simulink model "AvonGasTurbineDgTwin_fixed"  (R2024b)
settings: Solver=VariableStepAuto  StartTime=0  StopTime=7200  FixedStep=1  RelTol=1e-3  EnableMultiTasking=on
InitFcn:
  | warning off
model workspace (MAT data in the model file):
  FAULT_01_AirIntakeFilterFouling_enable = 1
  FAULT_02_CompBladeFouling_enable = 1
  FAULT_03_CompBladeDamage_enable = 1
  FAULT_04_CompSurgeStall_enable = 1
  FAULT_05_DiffuserDamage_enable = 1
  FAULT_06_IGVStuck_enable = 1
  FAULT_07_FuelPrssRegulatorStuck_enable = 1
  FAULT_08_FuelValveLeakage_enable = 1
  FAULT_09_FuelContamination_enable = 1
  FAULT_10_FuelLineBlockage_enable = 1
  FAULT_11_FuelPumpDegradation_enable = 1
  FAULT_12_FuelSupplyPressDrop_enable = 1
  FAULT_13_FGSupplyPressOscillation_enable = 1
  FAULT_14_FGValvePartialOpening_enable = 1
  FAULT_15_FGValveActuatorDelay_enable = 1
  FAULT_15_FuelPressReg_enable = 0
  FAULT_16_CombLinerDamage_enable = 1
  FAULT_16_FuelValveLeak_enable = 0
  FAULT_17_FuelNozzleClogging_enable = 1
  FAULT_18_CombustionFlameOscillation_enable = 1
  FAULT_19_CombustionInstability_enable = 1
  FAULT_20_HotGasPathTempIncrease_enable = 1
  FAULT_21_GGTurbFouling_enable = 1
  FAULT_22_GGTurbBladeDamage_enable = 1
  FAULT_23_GGNozzleBlockage_enable = 1
  FAULT_24_GGSealDegradation_enable = 1
  FAULT_25_GGInletPressureLoss_enable = 1
  FAULT_26_PTFouling_enable = 1
  FAULT_27_PTBladeDamage_enable = 1
  FAULT_28_PTNozzleDamage_enable = 1
  FAULT_29_PTSealDegradation_enable = 1
  FAULT_30_PTBearingWear_enable = 1
  FAULT_31_PTPowerLoss_enable = 1
  FAULT_32_PTStackBlockage_enable = 1
  FAULT_33_SensorEnhancement_enable = 1
  FAULT_34_SensorDegradation_enable = 1
  FAULT_35_SensorEnhanceStep_enable = 1
  FAULT_36_SensorDegradeStep_enable = 1
  FAULT_37_SensorFreez_enable = 1
  FAULT_38_GGSpeedSensor_enable = 1
  FAULT_39_PTSpeedSensor_enable = 1
  FAULT_40_FGSensorOffset_enable = 1
  FAULT_41_FGSensorDrift_enable = 1
  FAULT_42_ControlLoopOscillation_enable = 1
  GOV_GG_BASELINE = 10
  GOV_GG_DROOP_PCT = 0.04
  GOV_PT_BASELINE = 10
  GOV_PT_DROOP_PCT = 0.04
  SW_Manual_Switch1_enable = 1
  SW_Manual_Switch2_enable = 1
  SW_Manual_Switch3_enable = 1
  SW_Manual_Switch4_enable = 1
  SW_Manual_Switch_enable = 1
undefined symbols (not defined in the file or in its folder): ENV_ambient_moisture_pct, ENV_comp_inlet_press_kPa, ENV_FG_pressure_kPa, ENV_FG_temp_C, SP_POWER_CMD
libraries: slpidlib x3, simulink x2
(part 3 of 4)

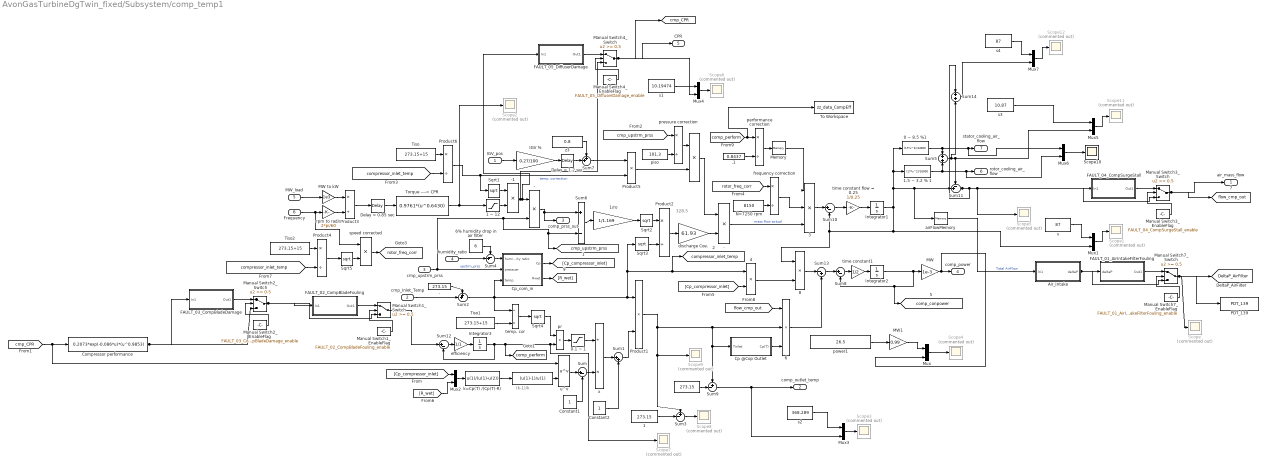
== system AvonGasTurbineDgTwin_fixed/Subsystem/comp_temp1 ==
  note: (k-1)/k
  note: 328.5
  IGV_pos : Inport
  cmp_Inlet_Temp : Inport  Port=2
  cmp_upstrm_prss : Inport  Port=3
  humidity_ratio : Inport  Port=4
  MW_load : Inport  Port=5
  Frequency : Inport  Port=6
  " " : Fcn  Expr=(u(1)-1)/u(1)
  "    " : Constant  Value=273.15
  "     " : Product  RndMeth=Zero
  "    1" : Constant  Value=273.15
  " 1.5 ~ 3.2 % 1" : Fcn  Expr=(17*u^2)/16000  SampleTime=1
  " 3" : Product  Inputs=3  RndMeth=Zero
  " 4" : Product  RndMeth=Zero
  " 6" : Product  Inputs=3  RndMeth=Zero
  " 8" : Product  RndMeth=Zero
  - : Product  RndMeth=Zero
  -1 : Product  RndMeth=Zero
  . : Constant  Value=273.15
  ". " : Product  RndMeth=Zero
  .1 : Constant  Value=0.8437
  0 ~ 8.5 %1 : Fcn  Expr=(17*u^2)/44000  SampleTime=1
  0.1 ~ 1 : Saturate  UpperLimit=1  LowerLimit=0.1
  1 ~ 12 : Saturate  UpperLimit=20  LowerLimit=1
  1/ro : Gain  Gain=1/1.169
  6% humidity drop in air filter : Constant  Value=6
  Air_Intake : Subsystem
  "Compressor performance " : Fcn  Expr=0.2073*exp(-0.086*u)*(u^0.9853)
  Constant1 : Constant
  Constant2 : Constant
  Cp @Cop Outlet : Subsystem
  Cp_com_in : Subsystem
  Delay = 0.85 sec : TransportDelay  DelayTime=0.85  InitialOutput=10.706
  Delay = 1.2 sec : TransportDelay  DelayTime=1.2  InitialOutput=0.27
  FAULT_01_AirIntakeFilterFouling : Subsystem
  FAULT_02_CompBladeFouling : Subsystem
  FAULT_03_CompBladeDamage : Subsystem
  FAULT_04_CompSurgeStall : Subsystem
  FAULT_05_DiffuserDamage : Subsystem
  IGV % : Gain  Gain=0.27/100
  Integrator1 : Integrator  InitialCondition=87  LimitOutput=on  UpperSaturationLimit=140  LowerSaturationLimit=1
  Integrator2 : Integrator  InitialCondition=28000  LimitOutput=on  UpperSaturationLimit=32000  LowerSaturationLimit=10
  Integrator3 : Integrator  InitialCondition=0.6  LimitOutput=on  UpperSaturationLimit=1  LowerSaturationLimit=0
  MW : Gain  Gain=1e-3
  MW to kW : Gain  Gain=1e3
  MW1 : Gain  Gain=0.99
  Manual Switch1_EnableFlag : Constant  Value=FAULT_02_CompBladeFouling_enable
  Manual Switch1_Switch : Switch  Threshold=0.5  SaturateOnIntegerOverflow=off  InputSameDT=off
  Manual Switch2_EnableFlag : Constant  Value=FAULT_03_CompBladeDamage_enable
  Manual Switch2_Switch : Switch  Threshold=0.5  SaturateOnIntegerOverflow=off  InputSameDT=off
  Manual Switch3_EnableFlag : Constant  Value=FAULT_04_CompSurgeStall_enable
  Manual Switch3_Switch : Switch  Threshold=0.5  SaturateOnIntegerOverflow=off  InputSameDT=off
  Manual Switch4_EnableFlag : Constant  Value=FAULT_05_DiffuserDamage_enable
  Manual Switch4_Switch : Switch  Threshold=0.5  SaturateOnIntegerOverflow=off  InputSameDT=off
  Manual Switch7_EnableFlag : Constant  Value=FAULT_01_AirIntakeFilterFouling_enable
  Manual Switch7_Switch : Switch  Threshold=0.5  SaturateOnIntegerOverflow=off  InputSameDT=off
  Memory : Memory  InitialCondition=1.5
  Mux{,1..7} (8 alike) : Mux  Inputs=2
  N=7250 rpm : Constant  Value=8150
  PDT_139 : ToWorkspace  VariableName=PDT_139  SampleTime=0.2
  Product1 : Product  RndMeth=Zero
  Product{2..4,6} (4 alike) : Product  Inputs=*/  RndMeth=Zero
  Product5 : Product  RndMeth=Zero
  Scope{,1..9,11..12} (12 alike) : Scope  Commented=on
  Scope10 : Scope
  Sqrt{1..5} (5 alike) : Sqrt
  Sum{,8,10,12} (4 alike) : Sum  Inputs=|+-
  Sum1 : Sum  Inputs=|++
  Sum11 : Sum  Inputs=-+|
  Sum13 : Sum  Inputs=|-+
  Sum14 : Sum
  Sum2 : Sum  Inputs=++|
  Sum3 : Sum  Inputs=+-|
  Sum4 : Sum  Inputs=-+|
  Sum5 : Sum
  Sum6 : Sum  Inputs=+-
  Sum7 : Sum  Inputs=++|
  Sum9 : Sum  Inputs=+-|
  Tiso : Constant  Value=273.15+15
  Tiso1 : Constant  Value=273.15+15
  Tiso2 : Constant  Value=273.15+15
  To Workspace : ToWorkspace  VariableName=zz_data_CompEff  SampleTime=0.2
  Torque ----> CPR : Fcn  Expr=0.9761*(u^0.6430)
  airFlowMemory : Memory  InitialCondition=80
  "discharge Coe. " : Gain  Gain=61.93
  efficiency : Gain  Gain=1/1
  frequency correction : Product  Inputs=*/  RndMeth=Zero
  k=Cp(T) /(Cp(T)-R) : Fcn  Expr=u(1)/(u(1)-u(2))
  performance correction : Product  Inputs=*/  RndMeth=Zero
  piso : Constant  Value=101.3
  power1 : Constant  Value=26.5
  "pr " : Product  RndMeth=Zero
  pressure correction : Product  Inputs=*/  RndMeth=Zero
  rpm to rad/s : Gain  Gain=2*pi/60
  s : Constant  Value=87
  s1 : Constant  Value=10.19474
  s2 : Constant  Value=368.289
  s3 : Constant  Value=10.87
  s4 : Constant  Value=87
  speed corrected : Product  RndMeth=Zero
  temp. cor : Product  Inputs=/*  RndMeth=Zero
  time constant flow = 0.25 : Gain  Gain=1/0.25
  time constant1 : Gain  Gain=1/2
  u^v : Math  Operator=pow  SignedPower=on
  x : Product  Inputs=/*  RndMeth=Zero
  z3 : Constant  Value=0.8
  air_mass_flow : Outport
  comp_outlet_temp : Outport  Port=2
  comp_prss_out : Outport  Port=3
  comp_power : Outport  Port=4
  CPR : Outport  Port=5
  rotor_cooling_air_flow : Outport  Port=6
  stator_cooling_air_flow : Outport  Port=7
  tag scope: DeltaP_AirFilter=global, cmp_CPR=global, cmp_upstrm_prss=global, comp_conpower=global, comp_perform=global, compressor_inlet_temp=global, flow_cmp_out=global, rotor_freq_corr=global
  wires:
  [cmp_CPR] -> "Compressor performance "/1, u^v/1
  " "/1 -> u^v/2
  u^v/1 -> Sum/1
  Sum/1 -> x/2
  Constant2/1 -> Sum1/2
  Sum1/1 -> Product1/2
  Sum2/1 -> Cp_com_in/3(temp.), Product1/1, Sqrt3/1, [compressor_inlet_temp], " 4"/1, temp. cor/1
  x/1 -> Sum1/1
  Constant1/1 -> Sum/2
  cmp_upstrm_prss/1 -> Cp_com_in/2(pressuer), -/2, [cmp_upstrm_prss], Sum6/2  "upstrm_prss"
  cmp_Inlet_Temp/1 -> Sum2/2
  0.1 ~ 1/1 -> x/1
  k=Cp(T) /(Cp(T)-R)/1 -> " "/1
  Cp_com_in/1(Cp) -> [Cp_compressor_inlet]
  Sum4/1 -> Cp_com_in/1(humidity ratio)
  humidity_ratio/1 -> Sum4/2
  6% humidity drop in air filter/1 -> Sum4/1
  -/1 -> comp_prss_out/1, Sum6/1
  Frequency/1 -> speed corrected/1, rpm to rad/s/1
  Sum6/1 -> 1/ro/1
  1/ro/1 -> Sqrt2/1
  Sqrt3/1 -> Product2/2
  Product2/1 -> "discharge Coe. "/1
  Sqrt2/1 -> Product2/1
  IGV_pos/1 -> IGV %/1
  piso/1 -> pressure correction/2
  [cmp_upstrm_prss] -> pressure correction/1
  Product5/1 -> "     "/2
  "discharge Coe. "/1 -> ". "/2
  "     "/1 -> ". "/1
  ". "/1 -> " 3"/3  "mass flow actual"
  Product6/1 -> Product5/2, Sqrt1/1  "temp. correction"
  Tiso/1 -> Product6/1
  [compressor_inlet_temp] -> Product6/2
  pressure correction/1 -> "     "/1
  1 ~ 12/1 -> -1/2
  N=7250 rpm/1 -> frequency correction/2
  [rotor_freq_corr] -> frequency correction/1
  frequency correction/1 -> " 3"/2
  " 3"/1 -> Sum10/1
  [Cp_compressor_inlet] -> " 4"/2
  Sum10/1 -> time constant flow = 0.25/1
  time constant flow = 0.25/1 -> Integrator1/1
  " 4"/1 -> " 8"/2
  " 8"/1 -> Sum13/1
  Sqrt1/1 -> -1/1
  Sum7/1 -> Product5/1
  z3/1 -> Sum7/1
  IGV %/1 -> Delay = 1.2 sec/1
  Delay = 1.2 sec/1 -> Sum7/2
  MW_load/1 -> MW to kW/1
  Cp_com_in/2(Rwet) -> [R_wet]
  Mux2/1 -> k=Cp(T) /(Cp(T)-R)/1
  [Cp_compressor_inlet] -> Mux2/1
  [R_wet] -> Mux2/2
  Sum8/1 -> time constant1/1
  time constant1/1 -> Integrator2/1
  Sum13/1 -> Sum8/1
  ./1 -> Sum2/1
  Tiso1/1 -> temp. cor/2
  temp. cor/1 -> Sqrt4/1
  "pr "/1 -> 0.1 ~ 1/1
  Sum12/1 -> efficiency/1
  efficiency/1 -> Integrator3/1
  Sqrt4/1 -> "pr "/1
  Torque ----> CPR/1 -> Scope2/1, 1 ~ 12/1
  MW to kW/1 -> Product3/1
  rpm to rad/s/1 -> Product3/2
  Integrator3/1 -> [comp_perform], Scope7/1, "pr "/2, Sum12/2
  Integrator2/1 -> MW/1, [comp_conpower], Sum8/2
  Product1/1 -> " 6"/2, Cp @Cop Outlet/1(Tinlet), Sum9/1, Scope9/1, Sum3/1
  Cp @Cop Outlet/1(Cp(T)) -> " 6"/3
  " 6"/1 -> Sum13/2
  "    "/1 -> Sum9/2
  Tiso2/1 -> Product4/1
  [compressor_inlet_temp] -> Product4/2
  speed corrected/1 -> [rotor_freq_corr]
  Product4/1 -> Sqrt5/1
  Sqrt5/1 -> speed corrected/2
  [flow_cmp_out] -> " 6"/1
  Mux/1 -> Scope4/1
  Sum11/1 -> Sum14/1, Scope5/1, FAULT_04_CompSurgeStall/1(In1), Manual Switch3_Switch/3
  0 ~ 8.5 %1/1 -> Sum5/1, Mux6/1, stator_cooling_air_flow/1
  Integrator1/1 -> Mux1/2, " 8"/1, Sum10/2, airFlowMemory/1, Sum11/2, " 1.5 ~ 3.2 % 1"/1, 0 ~ 8.5 %1/1
  Mux1/1 -> Scope1/1
  s/1 -> Mux1/1
  Product3/1 -> Delay = 0.85 sec/1
  Delay = 0.85 sec/1 -> Torque ----> CPR/1
  power1/1 -> MW1/1
  Mux3/1 -> Scope3/1
  s2/1 -> Mux3/1
  MW/1 -> Mux/2, comp_power/1
  Mux4/1 -> Scope6/1
  s1/1 -> Mux4/1
  -1/1 -> -/1, FAULT_05_DiffuserDamage/1(In1), Manual Switch4_Switch/3
  Sum9/1 -> Mux3/2, comp_outlet_temp/1
  "    1"/1 -> Sum3/2
  Sum3/1 -> Scope8/1
  MW1/1 -> Mux/1
  Sum5/1 -> Sum14/2, Sum11/1, Mux5/2
  Mux5/1 -> Scope11/1
  s3/1 -> Mux5/1
  Mux6/1 -> Scope10/1
  " 1.5 ~ 3.2 % 1"/1 -> Sum5/2, Mux6/2, rotor_cooling_air_flow/1
  Sum14/1 -> Mux7/2
  Mux7/1 -> Scope12/1
  s4/1 -> Mux7/1
  performance correction/1 -> Memory/1
  .1/1 -> performance correction/2
  [comp_perform] -> To Workspace/1, performance correction/1
  Memory/1 -> " 3"/1
  "Compressor performance "/1 -> FAULT_03_CompBladeDamage/1(In1), Manual Switch2_Switch/3
  airFlowMemory/1 -> Air_Intake/1(In1)  "Total AirFlow"
  Air_Intake/1(deltaP) -> FAULT_01_AirIntakeFilterFouling/1(deltaP), Manual Switch7_Switch/3
  FAULT_02_CompBladeFouling/1(Out1) -> Manual Switch1_Switch/1
  Manual Switch1_EnableFlag/1 -> Manual Switch1_Switch/2
  Manual Switch1_Switch/1 -> Sum12/1
  FAULT_03_CompBladeDamage/1(Out1) -> Manual Switch2_Switch/1
  Manual Switch2_EnableFlag/1 -> Manual Switch2_Switch/2
  Manual Switch2_Switch/1 -> Manual Switch1_Switch/3, FAULT_02_CompBladeFouling/1(In1)
  FAULT_04_CompSurgeStall/1(Out1) -> Manual Switch3_Switch/1
  Manual Switch3_EnableFlag/1 -> Manual Switch3_Switch/2
  Manual Switch3_Switch/1 -> air_mass_flow/1, [flow_cmp_out]
  FAULT_05_DiffuserDamage/1(Out1) -> Manual Switch4_Switch/1
  Manual Switch4_EnableFlag/1 -> Manual Switch4_Switch/2
  Manual Switch4_Switch/1 -> [cmp_CPR], CPR/1, Mux4/2
  FAULT_01_AirIntakeFilterFouling/1(Out1) -> Manual Switch7_Switch/1
  Manual Switch7_EnableFlag/1 -> Manual Switch7_Switch/2
  Manual Switch7_Switch/1 -> [DeltaP_AirFilter], PDT_139/1, Scope/1

== system AvonGasTurbineDgTwin_fixed/Subsystem2/FAULT_42_ControlLoopOscillation ==
  In1 : Inport
  FAULT_42_multiplier : FromWorkspace  VariableName=FAULT_42_multiplier  SampleTime=-1
  Mux : Mux  Inputs=2
  Product : Product
  Scope{,1..3} (4 alike) : Scope  Commented=on
  Out1 : Outport
  wires:
  FAULT_42_multiplier/1 -> Product/1, Scope/1
  In1/1 -> Scope1/1, Mux/2, Product/2
  Product/1 -> Mux/1, Scope2/1, Out1/1
  Mux/1 -> Scope3/1

== system AvonGasTurbineDgTwin_fixed/Subsystem/Combustor1/FAULT_16_CombLinerDamage ==
  air_flow : Inport
  FAULT_16_multiplier : FromWorkspace  VariableName=FAULT_16_multiplier  SampleTime=-1
  Mux : Mux  Inputs=2
  Product : Product
  Scope{,1..3} (4 alike) : Scope  Commented=on
  Out1 : Outport
  wires:
  FAULT_16_multiplier/1 -> Product/1, Scope/1
  air_flow/1 -> Scope1/1, Mux/2, Product/2
  Product/1 -> Mux/1, Scope2/1, Out1/1
  Mux/1 -> Scope3/1

== system AvonGasTurbineDgTwin_fixed/Subsystem/Combustor1/FAULT_17_FuelNozzleClogging ==
  FG flow : Inport
  FAULT_17_multiplier : FromWorkspace  VariableName=FAULT_17_multiplier  SampleTime=-1
  Mux : Mux  Inputs=2
  Product : Product
  Scope{,1..3} (4 alike) : Scope  Commented=on
  Out1 : Outport
  wires:
  FAULT_17_multiplier/1 -> Product/1, Scope/1
  FG flow/1 -> Scope1/1, Mux/2, Product/2
  Product/1 -> Mux/1, Scope2/1, Out1/1
  Mux/1 -> Scope3/1

== system AvonGasTurbineDgTwin_fixed/Subsystem/Combustor1/FAULT_18_CombustionFlameOscillation ==
  temp chamber 1 : Inport
  FAULT_18_multiplier : FromWorkspace  VariableName=FAULT_18_multiplier  SampleTime=-1
  Mux : Mux  Inputs=2
  Product : Product
  Scope{,1..3} (4 alike) : Scope  Commented=on
  Out1 : Outport
  wires:
  FAULT_18_multiplier/1 -> Product/1, Scope/1
  temp chamber 1/1 -> Scope1/1, Mux/2, Product/2
  Product/1 -> Mux/1, Scope2/1, Out1/1
  Mux/1 -> Scope3/1

== system AvonGasTurbineDgTwin_fixed/Subsystem/Combustor1/FAULT_19_CombustionInstability ==
  In1 : Inport
  FAULT_19_multiplier : FromWorkspace  VariableName=FAULT_19_multiplier  SampleTime=-1
  Mux : Mux  Inputs=2
  Product : Product
  Scope{,1..3} (4 alike) : Scope  Commented=on
  Out1 : Outport
  wires:
  FAULT_19_multiplier/1 -> Product/1, Scope/1
  In1/1 -> Scope1/1, Mux/2, Product/2
  Product/1 -> Mux/1, Scope2/1, Out1/1
  Mux/1 -> Scope3/1

== system AvonGasTurbineDgTwin_fixed/Subsystem/Combustor1/FAULT_20_HotGasPathTempIncrease ==
  In1 : Inport
  FAULT_20_multiplier : FromWorkspace  VariableName=FAULT_20_multiplier  SampleTime=-1
  Mux : Mux  Inputs=2
  Product : Product
  Scope{,1..3} (4 alike) : Scope  Commented=on
  Out1 : Outport
  wires:
  FAULT_20_multiplier/1 -> Product/1, Scope/1
  In1/1 -> Scope1/1, Mux/2, Product/2
  Product/1 -> Mux/1, Scope2/1, Out1/1
  Mux/1 -> Scope3/1

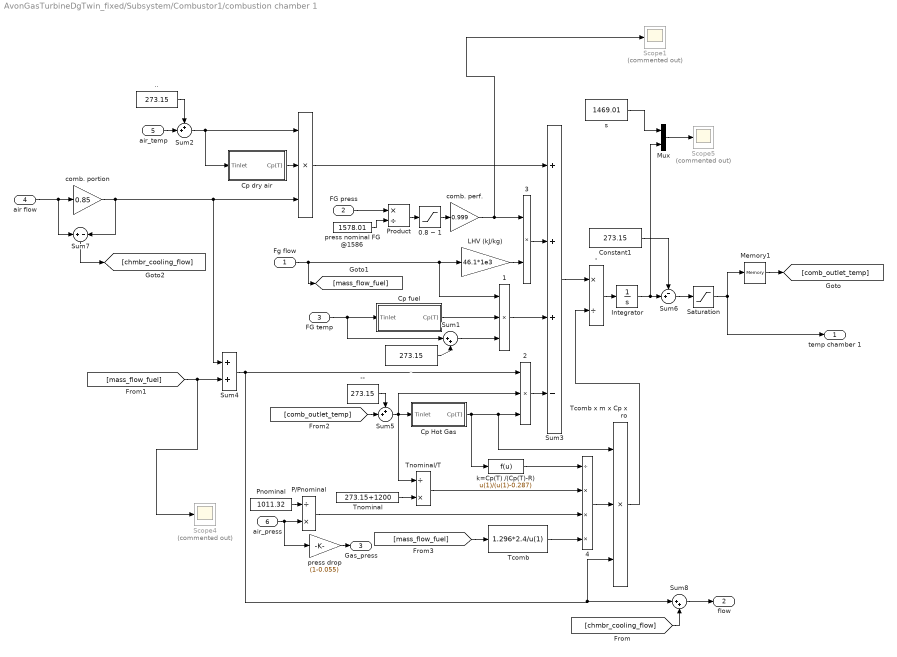
== system AvonGasTurbineDgTwin_fixed/Subsystem/Combustor1/combustion chamber 1 ==
  Fg flow : Inport
  FG press : Inport  Port=2
  FG temp : Inport  Port=3
  air flow : Inport  Port=4
  air_temp : Inport  Port=5
  air_press : Inport  Port=6
  "     " : Product  Inputs=3  RndMeth=Zero
  "     1" : Product  Inputs=3  RndMeth=Zero
  "     2" : Product  Inputs=3  RndMeth=Zero
  "     3" : Product  RndMeth=Zero
  "     4" : Product  Inputs=/***  RndMeth=Zero
  " Cp dry air " : Subsystem
  - : Product  Inputs=*/  RndMeth=Zero
  -- : Constant  Value=273.15
  . : Constant  Value=273.15
  .. : Constant  Value=273.15
  0.8 ~ 1 : Saturate  UpperLimit=1  LowerLimit=0.8
  Constant1 : Constant  Value=273.15
  "Cp Hot Gas " : Subsystem
  Cp fuel : Subsystem
  Integrator : Integrator  InitialCondition=780+273.15  LimitOutput=on  UpperSaturationLimit=2000  LowerSaturationLimit=780+273.15
  "LHV (kJ/kg) " : Gain  Gain=46.1*1e3
  Memory1 : Memory  InitialCondition=780
  Mux : Mux  Inputs=2
  P/Pnominal : Product  Inputs=/*  RndMeth=Zero
  Pnominal : Constant  Value=1011.32
  Product : Product  Inputs=*/
  Saturation : Saturate  UpperLimit=1400  LowerLimit=350
  Scope1 : Scope  Commented=on
  Scope4 : Scope  Commented=on
  Scope5 : Scope  Commented=on
  Sum1 : Sum  Inputs=|++
  Sum2 : Sum  Inputs=++|
  Sum3 : Sum  Inputs=+++-
  Sum4 : Sum  Inputs=2
  Sum5 : Sum  Inputs=++|
  Sum6 : Sum  Inputs=-+|
  Sum7 : Sum  Inputs=+-
  Sum8 : Sum  Inputs=|++
  Tcomb : Fcn  Expr=1.296*2.4/u(1)  SampleTime=1
  Tcomb x m x Cp x ro : Product  Inputs=3  RndMeth=Zero
  Tnominal : Constant  Value=273.15+1200
  Tnominal/T : Product  Inputs=/*  RndMeth=Zero
  comb. perf. : Gain  Gain=0.999
  comb. portion : Gain  Gain=0.85
  k=Cp(T) /(Cp(T)-R) : Fcn  Expr=u(1)/(u(1)-0.287)
  press drop : Gain  Gain=(1-0.055)  SampleTime=1
  press nominal FG @1586 : Constant  Value=1578.01
  s : Constant  Value=1469.01
  temp chamber 1 : Outport
  flow : Outport  Port=2
  Gas_press : Outport  Port=3
  wires:
  " Cp dry air "/1(Cp(T)) -> "     "/2
  ../1 -> Sum2/1
  Sum2/1 -> " Cp dry air "/1(Tinlet), "     "/1
  FG press/1 -> Product/1
  FG temp/1 -> Sum1/1, Cp fuel/1(Tinlet)
  Sum3/1 -> -/1
  Fg flow/1 -> "     1"/1, "LHV (kJ/kg) "/1, [mass_flow_fuel]
  Sum1/1 -> "     1"/3
  Cp fuel/1(Cp(T)) -> "     1"/2
  "     "/1 -> Sum3/1
  Memory1/1 -> [comb_outlet_temp]
  "     1"/1 -> Sum3/3
  ./1 -> Sum1/2
  "     2"/1 -> Sum3/4
  Tnominal/1 -> Tnominal/T/2
  Sum5/1 -> "     2"/2, "Cp Hot Gas "/1(Tinlet), Tnominal/T/1
  Constant1/1 -> Sum6/1
  Integrator/1 -> Mux/2, Sum6/2
  Sum6/1 -> Saturation/1
  "LHV (kJ/kg) "/1 -> "     3"/2
  Tcomb x m x Cp x ro/1 -> -/2
  Tnominal/T/1 -> "     4"/2
  [mass_flow_fuel] -> Scope4/1, Sum4/2
  "Cp Hot Gas "/1(Cp(T)) -> k=Cp(T) /(Cp(T)-R)/1, "     2"/3, Tcomb x m x Cp x ro/1
  --/1 -> Sum5/1
  Pnominal/1 -> P/Pnominal/1
  air_press/1 -> press drop/1, P/Pnominal/2
  "     4"/1 -> Tcomb x m x Cp x ro/2
  k=Cp(T) /(Cp(T)-R)/1 -> "     4"/1
  [comb_outlet_temp] -> Sum5/2
  P/Pnominal/1 -> "     4"/3
  air_temp/1 -> Sum2/2
  -/1 -> Integrator/1
  Saturation/1 -> temp chamber 1/1, Memory1/1
  s/1 -> Mux/1
  Sum4/1 -> "     2"/1, Sum8/1, Tcomb x m x Cp x ro/3
  Mux/1 -> Scope5/1
  press drop/1 -> Gas_press/1
  press nominal FG @1586/1 -> Product/2
  Product/1 -> 0.8 ~ 1/1
  0.8 ~ 1/1 -> comb. perf./1
  comb. perf./1 -> "     3"/1, Scope1/1
  "     3"/1 -> Sum3/2
  [mass_flow_fuel] -> Tcomb/1
  Tcomb/1 -> "     4"/4
  air flow/1 -> Sum7/1, comb. portion/1
  comb. portion/1 -> Sum7/2, "     "/3, Sum4/1
  Sum8/1 -> flow/1
  [chmbr_cooling_flow] -> Sum8/2
  Sum7/1 -> [chmbr_cooling_flow]

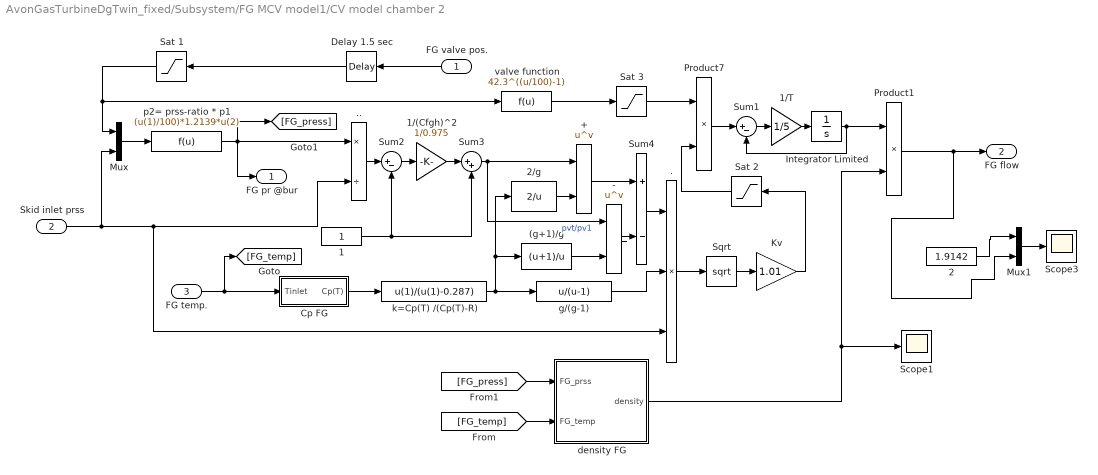
== system AvonGasTurbineDgTwin_fixed/Subsystem/FG MCV model1/CV model chamber 2 ==
  FG valve pos. : Inport
  Skid inlet prss : Inport  Port=2
  FG temp. : Inport  Port=3
  "  (g+1)/g" : Fcn  Expr=(u+1)/u
  "  Sqrt  " : Sqrt
  " k=Cp(T) /(Cp(T)-R) " : Fcn  Expr=u(1)/(u(1)-0.287)
  + : Math  Operator=pow  SignedPower=on
  - : Math  Operator=pow  SignedPower=on
  . : Product  Inputs=3  RndMeth=Zero
  .. : Product  Inputs=*/  RndMeth=Zero
  1 : Constant
  1/(Cfgh)^2 : Gain  Gain=1/0.975
  1/T : Gain  Gain=1/5
  2 : Constant  Value=1.9142
  2/g : Fcn  Expr=2/u
  Cp FG : Subsystem
  Delay 1.5 sec : TransportDelay  DelayTime=1.5  InitialOutput=30
  Integrator Limited : Integrator  InitialCondition=1.9  LimitOutput=on  UpperSaturationLimit=5  LowerSaturationLimit=0.01
  Kv : Gain  Gain=1.01
  Mux : Mux  Inputs=2
  Mux1 : Mux  Inputs=2
  Product1 : Product  RndMeth=Zero
  Product7 : Product  RndMeth=Zero
  Sat 1 : Saturate  UpperLimit=100  LowerLimit=0.01
  Sat 2 : Saturate  UpperLimit=300  LowerLimit=0.001
  Sat 3 : Saturate  UpperLimit=1  LowerLimit=0.01
  Scope1 : Scope
  Scope3 : Scope
  Sum1 : Sum  Inputs=|+-
  Sum2 : Sum  Inputs=|+-
  Sum3 : Sum  Inputs=|++
  Sum4 : Sum  Inputs=+-
  density FG : Subsystem
  g/(g-1) : Fcn  Expr=u/(u-1)
  p2= prss-ratio * p1 : Fcn  Expr=(u(1)/100)*1.2139*u(2)  SampleTime=1
  valve function : Fcn  Expr=42.3^((u/100)-1)  SampleTime=1
  FG pr @bur : Outport
  FG flow : Outport  Port=2
  wires:
  Sat 2/1 -> Product7/2
  Sum3/1 -> +/1, -/1  "pvt/pv1"
  Sum4/1 -> ./1
  "  Sqrt  "/1 -> Kv/1
  ../1 -> Sum2/1
  Skid inlet prss/1 -> ../2, ./3, Mux/2
  2/g/1 -> +/2
  1/(Cfgh)^2/1 -> Sum3/1
  Sum2/1 -> 1/(Cfgh)^2/1
  FG temp./1 -> [FG_temp], Cp FG/1(Tinlet)
  "  (g+1)/g"/1 -> -/2
  -/1 -> Sum4/2
  " k=Cp(T) /(Cp(T)-R) "/1 -> g/(g-1)/1, "  (g+1)/g"/1, 2/g/1
  g/(g-1)/1 -> ./2
  p2= prss-ratio * p1/1 -> [FG_press], ../1, FG pr @bur/1
  +/1 -> Sum4/1
  1/1 -> Sum3/2, Sum2/2
  Cp FG/1(Cp(T)) -> " k=Cp(T) /(Cp(T)-R) "/1
  Mux/1 -> p2= prss-ratio * p1/1
  valve function/1 -> Sat 3/1
  FG valve pos./1 -> Delay 1.5 sec/1
  Delay 1.5 sec/1 -> Sat 1/1
  Sat 1/1 -> Mux/1, valve function/1
  Sat 3/1 -> Product7/1
  Kv/1 -> Sat 2/1
  Sum1/1 -> 1/T/1
  1/T/1 -> Integrator Limited/1
  Integrator Limited/1 -> Product1/1, Sum1/2
  ./1 -> "  Sqrt  "/1
  Product7/1 -> Sum1/1
  [FG_temp] -> density FG/2(FG_temp)
  [FG_press] -> density FG/1(FG_prss)
  density FG/1(density) -> Scope1/1, Product1/2
  Mux1/1 -> Scope3/1
  Product1/1 -> Mux1/2, FG flow/1
  2/1 -> Mux1/1

== system AvonGasTurbineDgTwin_fixed/Subsystem/FG MCV model1/FAULT_07_FuelPrssRegulatorStuck ==
  main FG line prss : Inport
  FAULT_07_multiplier : FromWorkspace  VariableName=FAULT_07_multiplier  SampleTime=-1
  Mux : Mux  Inputs=2
  Product : Product
  Scope{,1..3} (4 alike) : Scope  Commented=on
  Out1 : Outport
  wires:
  FAULT_07_multiplier/1 -> Product/1, Scope/1
  main FG line prss/1 -> Scope1/1, Mux/2, Product/2
  Product/1 -> Mux/1, Scope2/1, Out1/1
  Mux/1 -> Scope3/1

== system AvonGasTurbineDgTwin_fixed/Subsystem/FG MCV model1/FAULT_08_FuelValveLeakage ==
  In1 : Inport
  FAULT_08_multiplier : FromWorkspace  VariableName=FAULT_08_multiplier  SampleTime=-1
  Mux : Mux  Inputs=2
  Product : Product
  Scope{,1..3} (4 alike) : Scope  Commented=on
  Out1 : Outport
  wires:
  FAULT_08_multiplier/1 -> Product/1, Scope/1
  In1/1 -> Scope1/1, Mux/2, Product/2
  Product/1 -> Mux/1, Scope2/1, Out1/1
  Mux/1 -> Scope3/1

== system AvonGasTurbineDgTwin_fixed/Subsystem/FG MCV model1/FAULT_09_FuelContamination ==
  In1 : Inport
  FAULT_09_multiplier : FromWorkspace  VariableName=FAULT_09_multiplier  SampleTime=-1
  Mux : Mux  Inputs=2
  Product : Product
  Scope{,1..3} (4 alike) : Scope  Commented=on
  Out1 : Outport
  wires:
  FAULT_09_multiplier/1 -> Product/1, Scope/1
  In1/1 -> Scope1/1, Mux/2, Product/2
  Product/1 -> Mux/1, Scope2/1, Out1/1
  Mux/1 -> Scope3/1

== system AvonGasTurbineDgTwin_fixed/Subsystem/FG MCV model1/FAULT_10_FuelLineBlockage ==
  In1 : Inport
  FAULT_10_multiplier : FromWorkspace  VariableName=FAULT_10_multiplier  SampleTime=-1
  Mux : Mux  Inputs=2
  Product : Product
  Scope{,1..3} (4 alike) : Scope  Commented=on
  Out1 : Outport
  wires:
  FAULT_10_multiplier/1 -> Product/1, Scope/1
  In1/1 -> Scope1/1, Mux/2, Product/2
  Product/1 -> Mux/1, Scope2/1, Out1/1
  Mux/1 -> Scope3/1

== system AvonGasTurbineDgTwin_fixed/Subsystem/FG MCV model1/FAULT_11_FuelPumpDegradation ==
  In1 : Inport
  FAULT_11_multiplier : FromWorkspace  VariableName=FAULT_11_multiplier  SampleTime=-1
  Mux : Mux  Inputs=2
  Product : Product
  Scope{,1..3} (4 alike) : Scope  Commented=on
  Out1 : Outport
  wires:
  FAULT_11_multiplier/1 -> Product/1, Scope/1
  In1/1 -> Scope1/1, Mux/2, Product/2
  Product/1 -> Mux/1, Scope2/1, Out1/1
  Mux/1 -> Scope3/1

== system AvonGasTurbineDgTwin_fixed/Subsystem/FG MCV model1/FAULT_12_FuelSupplyPressDrop ==
  In1 : Inport
  FAULT_12_multiplier : FromWorkspace  VariableName=FAULT_12_multiplier  SampleTime=-1
  Mux : Mux  Inputs=2
  Product : Product
  Scope{,1..3} (4 alike) : Scope  Commented=on
  Out1 : Outport
  wires:
  FAULT_12_multiplier/1 -> Product/1, Scope/1
  In1/1 -> Scope1/1, Mux/2, Product/2
  Product/1 -> Mux/1, Scope2/1, Out1/1
  Mux/1 -> Scope3/1

== system AvonGasTurbineDgTwin_fixed/Subsystem/FG MCV model1/FAULT_13_FGSupplyPressOscillation ==
  In1 : Inport
  FAULT_13_multiplier : FromWorkspace  VariableName=FAULT_13_multiplier  SampleTime=-1
  Mux : Mux  Inputs=2
  Product : Product
  Scope{,1..3} (4 alike) : Scope  Commented=on
  Out1 : Outport
  wires:
  FAULT_13_multiplier/1 -> Product/1, Scope/1
  In1/1 -> Scope1/1, Mux/2, Product/2
  Product/1 -> Mux/1, Scope2/1, Out1/1
  Mux/1 -> Scope3/1

== system AvonGasTurbineDgTwin_fixed/Subsystem/FG MCV model1/FAULT_16_FuelValveLeak ==
  FG flow : Inport
  FAULT_16_multiplier : FromWorkspace  VariableName=FAULT_16_multiplier  SampleTime=-1
  Mux : Mux  Inputs=2
  Product : Product
  Scope{,1..3} (4 alike) : Scope  Commented=on
  Out1 : Outport
  wires:
  FAULT_16_multiplier/1 -> Product/1, Scope/1
  FG flow/1 -> Scope1/1, Mux/2, Product/2
  Product/1 -> Mux/1, Scope2/1, Out1/1
  Mux/1 -> Scope3/1

== system AvonGasTurbineDgTwin_fixed/Subsystem/FG MCV model1/Subsystem1 ==
  gas prss : Inport
  FG temp. : Inport  Port=2
  FG flow : Inport  Port=3
  " 2 " : Constant  Value=2
  . : Product  Inputs=3  RndMeth=Zero
  2 : Constant  Value=2
  Kf : Gain  Gain=16.8993
  Math Function5 : Math  Operator=pow  SignedPower=on
  Memory : Memory
  Sqrt : Sqrt
  Sqrt1 : Sqrt
  Sqrt2 : Sqrt
  Sum1 : Sum  Inputs=-+|
  Sum5 : Sum  Inputs=|++
  Sum9 : Sum  Inputs=|+-
  Z : Subsystem
  c4 : Constant  Value=273.15
  n flow exp. : Constant  Value=0.4835
  pressure drop 5 kPa : Constant  Value=5
  pw : Math  Operator=pow  SignedPower=on
  pw1 : Math  Operator=pow  SignedPower=on
  " FG skid inlet prss" : Outport
  skid temp : Outport  Port=2
  wires:
  pressure drop 5 kPa/1 -> Sum1/1
  Sum1/1 -> pw1/1
  Sqrt1/1 -> ./3
  Memory/1 -> Z/2(P)
  Sqrt/1 -> ./2
  Sum5/1 -> Z/1(T), Sqrt/1
  c4/1 -> Sum5/2
  Z/1(Z) -> Sqrt1/1
  Sqrt2/1 -> Memory/1, " FG skid inlet prss"/1
  Math Function5/1 -> ./1
  FG flow/1 -> Math Function5/1
  n flow exp./1 -> Math Function5/2
  pw/1 -> Sum9/2
  2/1 -> pw/2
  Sum9/1 -> Sqrt2/1
  pw1/1 -> Sum9/1
  Kf/1 -> pw/1
  ./1 -> Kf/1
  FG temp./1 -> Sum5/1, skid temp/1
  " 2 "/1 -> pw1/2
  gas prss/1 -> Sum1/2

== system AvonGasTurbineDgTwin_fixed/Subsystem/GasGenerator/Cp @ trb. input ==
  Tinlet : Inport
  Cp : Fcn  Expr=(3.355+5.75*1e-4*u(1)-1600*u(1)^(-2))*0.28714  SampleTime=1
  Cp(T) : Outport
  wires:
  Tinlet/1 -> Cp/1
  Cp/1 -> Cp(T)/1

== system AvonGasTurbineDgTwin_fixed/Subsystem/GasGenerator/Cp @ trb. output ==
  Tinlet : Inport
  Cp : Fcn  Expr=(3.355+5.75*1e-4*u(1)-1600*u(1)^(-2))*0.28714  SampleTime=1
  Cp(T) : Outport
  wires:
  Cp/1 -> Cp(T)/1
  Tinlet/1 -> Cp/1

== system AvonGasTurbineDgTwin_fixed/Subsystem/GasGenerator/FAULT_23_GGNozzleBlockage ==
  hot_gas_flow : Inport
  FAULT_23_multiplier : FromWorkspace  VariableName=FAULT_23_multiplier  SampleTime=-1
  Mux : Mux  Inputs=2
  Product : Product
  Scope{,1..3} (4 alike) : Scope  Commented=on
  Out1 : Outport
  wires:
  FAULT_23_multiplier/1 -> Product/1, Scope/1
  hot_gas_flow/1 -> Scope1/1, Mux/2, Product/2
  Product/1 -> Mux/1, Scope2/1, Out1/1
  Mux/1 -> Scope3/1

== system AvonGasTurbineDgTwin_fixed/Subsystem/GasGenerator/FAULT_24_GGSealDegradation ==
  rotor_cooling_air_flow : Inport
  FAULT_24_multiplier : FromWorkspace  VariableName=FAULT_24_multiplier  SampleTime=-1
  Mux : Mux  Inputs=2
  Product : Product
  Scope{,1..3} (4 alike) : Scope  Commented=on
  Out1 : Outport
  wires:
  FAULT_24_multiplier/1 -> Product/1, Scope/1
  rotor_cooling_air_flow/1 -> Scope1/1, Mux/2, Product/2
  Product/1 -> Mux/1, Scope2/1, Out1/1
  Mux/1 -> Scope3/1

== system AvonGasTurbineDgTwin_fixed/Subsystem/GasGenerator/FAULT_33_SensorEnhancement ==
  In1 : Inport
  FAULT_33_multiplier : FromWorkspace  VariableName=FAULT_33_multiplier  SampleTime=-1
  Mux : Mux  Inputs=2
  Product : Product
  Scope{,1..3} (4 alike) : Scope  Commented=on
  Out1 : Outport
  wires:
  FAULT_33_multiplier/1 -> Product/1, Scope/1
  In1/1 -> Scope1/1, Mux/2, Product/2
  Product/1 -> Mux/1, Scope2/1, Out1/1
  Mux/1 -> Scope3/1

== system AvonGasTurbineDgTwin_fixed/Subsystem/GasGenerator/FAULT_34_SensorDegradation ==
  In1 : Inport
  FAULT_34_multiplier : FromWorkspace  VariableName=FAULT_34_multiplier  SampleTime=-1
  Mux : Mux  Inputs=2
  Product : Product
  Scope{,1..3} (4 alike) : Scope  Commented=on
  Out1 : Outport
  wires:
  FAULT_34_multiplier/1 -> Product/1, Scope/1
  In1/1 -> Scope1/1, Mux/2, Product/2
  Product/1 -> Mux/1, Scope2/1, Out1/1
  Mux/1 -> Scope3/1

== system AvonGasTurbineDgTwin_fixed/Subsystem/GasGenerator/FAULT_35_SensorEnhanceStep ==
  In1 : Inport
  FAULT_35_multiplier : FromWorkspace  VariableName=FAULT_35_multiplier  SampleTime=-1
  Mux : Mux  Inputs=2
  Product : Product
  Scope{,1..3} (4 alike) : Scope  Commented=on
  Out1 : Outport
  wires:
  FAULT_35_multiplier/1 -> Product/1, Scope/1
  In1/1 -> Scope1/1, Mux/2, Product/2
  Product/1 -> Mux/1, Scope2/1, Out1/1
  Mux/1 -> Scope3/1

== system AvonGasTurbineDgTwin_fixed/Subsystem/GasGenerator/FAULT_36_SensorDegradeStep ==
  In1 : Inport
  FAULT_36_multiplier : FromWorkspace  VariableName=FAULT_36_multiplier  SampleTime=-1
  Mux : Mux  Inputs=2
  Product : Product
  Scope{,1..3} (4 alike) : Scope  Commented=on
  Out1 : Outport
  wires:
  FAULT_36_multiplier/1 -> Product/1, Scope/1
  In1/1 -> Scope1/1, Mux/2, Product/2
  Product/1 -> Mux/1, Scope2/1, Out1/1
  Mux/1 -> Scope3/1

== system AvonGasTurbineDgTwin_fixed/Subsystem/GasGenerator/FAULT_37_SensorFreez ==
  temp gas : Inport
  FAULT_37_multiplier : FromWorkspace  VariableName=FAULT_37_multiplier  SampleTime=-1
  Memory : Memory  InheritSampleTime=on
  Scope{,1..3} (4 alike) : Scope  Commented=on
  Switch : Switch  Criteria=u2 > Threshold  Threshold=0.5  SaturateOnIntegerOverflow=off  InputSameDT=off
  Out1 : Outport
  wires:
  FAULT_37_multiplier/1 -> Scope3/1, Switch/2
  temp gas/1 -> Scope2/1, Switch/1
  Memory/1 -> Scope/1, Switch/3
  Switch/1 -> Scope1/1, Out1/1, Memory/1

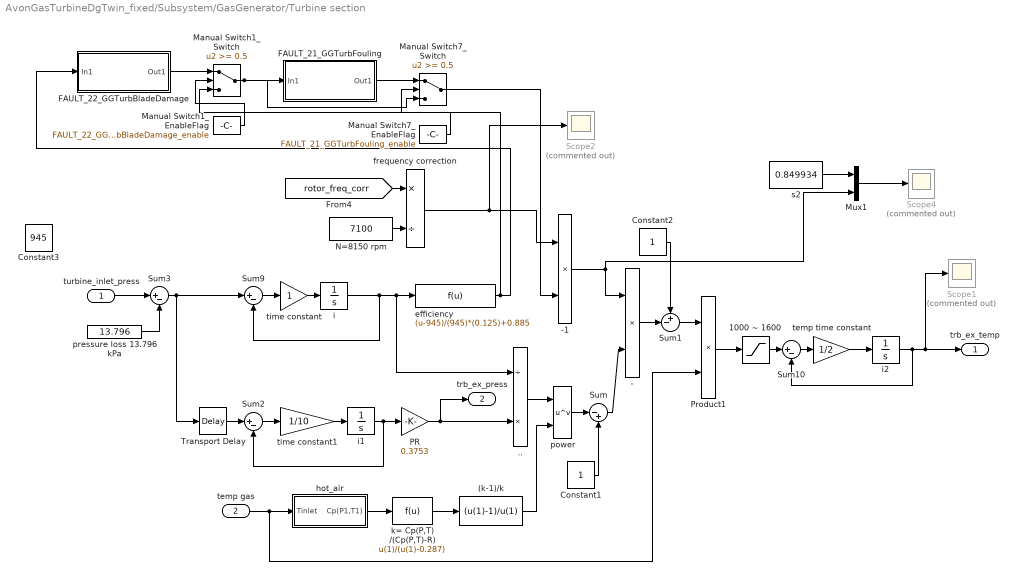
== system AvonGasTurbineDgTwin_fixed/Subsystem/GasGenerator/Turbine section ==
  turbine_inlet_press : Inport
  temp gas : Inport  Port=2
  (k-1)/k : Fcn  Expr=(u(1)-1)/u(1)
  - : Product  RndMeth=Zero
  -1 : Product  RndMeth=Zero
  .. : Product  Inputs=/*  RndMeth=Zero
  1000 ~ 1600 : Saturate  UpperLimit=2000  LowerLimit=400
  Constant1 : Constant
  Constant2 : Constant
  Constant3 : Constant  Value=945
  FAULT_21_GGTurbFouling : Subsystem
  FAULT_22_GGTurbBladeDamage : Subsystem
  Manual Switch1_EnableFlag : Constant  Value=FAULT_22_GGTurbBladeDamage_enable
  Manual Switch1_Switch : Switch  Threshold=0.5  SaturateOnIntegerOverflow=off  InputSameDT=off
  Manual Switch7_EnableFlag : Constant  Value=FAULT_21_GGTurbFouling_enable
  Manual Switch7_Switch : Switch  Threshold=0.5  SaturateOnIntegerOverflow=off  InputSameDT=off
  Mux1 : Mux  Inputs=2
  N=8150 rpm : Constant  Value=7100
  PR : Gain  Gain=0.3753
  Product1 : Product  RndMeth=Zero
  Scope1 : Scope  Commented=on
  Scope2 : Scope  Commented=on
  Scope4 : Scope  Commented=on
  Sum : Sum  Inputs=|-+
  Sum1 : Sum  Inputs=+-|
  Sum{2..3,9..10} (4 alike) : Sum  Inputs=|+-
  Transport Delay : TransportDelay  DelayTime=1.6  InitialOutput=941.9108
  efficiency : Fcn  Expr=(u-945)/(945)*(0.125)+0.885
  frequency correction : Product  Inputs=*/  RndMeth=Zero
  hot_air : Subsystem
  i : Integrator  InitialCondition=507  LimitOutput=on  UpperSaturationLimit=1100  LowerSaturationLimit=10
  i1 : Integrator  InitialCondition=507  LimitOutput=on  UpperSaturationLimit=1100  LowerSaturationLimit=500
  i2 : Integrator  InitialCondition=450+273.15  LimitOutput=on  UpperSaturationLimit=2000  LowerSaturationLimit=400
  k= Cp(P,T) /(Cp(P,T)-R) : Fcn  Expr=u(1)/(u(1)-0.287)
  power : Math  Operator=pow  SignedPower=on
  pressure loss 13.796 kPa : Constant  Value=13.796
  s2 : Constant  Value=0.849934
  temp time constant : Gain  Gain=1/2
  time constant : Gain
  time constant1 : Gain  Gain=1/10
  trb_ex_temp : Outport
  trb_ex_press : Outport  Port=2
  wires:
  i/1 -> Sum9/2, efficiency/1, ../1
  power/1 -> Sum/1
  Constant1/1 -> Sum/2
  -/1 -> Sum1/2
  Sum3/1 -> Sum9/1, Transport Delay/1
  k= Cp(P,T) /(Cp(P,T)-R)/1 -> (k-1)/k/1
  hot_air/1(Cp(P1,T1)) -> k= Cp(P,T) /(Cp(P,T)-R)/1
  (k-1)/k/1 -> power/2
  Sum/1 -> -/2
  Sum9/1 -> time constant/1
  time constant/1 -> i/1
  Sum10/1 -> temp time constant/1
  temp time constant/1 -> i2/1
  Product1/1 -> 1000 ~ 1600/1
  pressure loss 13.796 kPa/1 -> Sum3/2
  Constant2/1 -> Sum1/1
  Sum1/1 -> Product1/1
  temp gas/1 -> hot_air/1(Tinlet), Product1/2
  1000 ~ 1600/1 -> Sum10/1
  i2/1 -> Scope1/1, trb_ex_temp/1, Sum10/2
  Mux1/1 -> Scope4/1
  s2/1 -> Mux1/1
  -1/1 -> -/1, Mux1/2
  i1/1 -> Sum2/2, PR/1
  Sum2/1 -> time constant1/1
  time constant1/1 -> i1/1
  turbine_inlet_press/1 -> Sum3/1
  PR/1 -> trb_ex_press/1, ../2
  ../1 -> power/1
  Transport Delay/1 -> Sum2/1
  N=8150 rpm/1 -> frequency correction/2
  [rotor_freq_corr] -> frequency correction/1
  frequency correction/1 -> Scope2/1, -1/1
  efficiency/1 -> FAULT_22_GGTurbBladeDamage/1(In1), Manual Switch1_Switch/3
  FAULT_22_GGTurbBladeDamage/1(Out1) -> Manual Switch1_Switch/1
  Manual Switch1_EnableFlag/1 -> Manual Switch1_Switch/2
  Manual Switch1_Switch/1 -> FAULT_21_GGTurbFouling/1(In1), Manual Switch7_Switch/3
  FAULT_21_GGTurbFouling/1(Out1) -> Manual Switch7_Switch/1
  Manual Switch7_EnableFlag/1 -> Manual Switch7_Switch/2
  Manual Switch7_Switch/1 -> -1/2

== system AvonGasTurbineDgTwin_fixed/Subsystem/GasGenerator/cooling 1 ==
  cooling_air_temp : Inport
  cooling_air_flow : Inport  Port=2
  hot_gas_flow : Inport  Port=3
  hot_gas_temp : Inport  Port=4
  "     1" : Product  RndMeth=Zero
  "     2" : Product  Inputs=3  RndMeth=Zero
  "     4" : Product  Inputs=3  RndMeth=Zero
  . : Product  Inputs=*/  RndMeth=Zero
  Cp Temp : Subsystem
  Cp Temp air : Subsystem
  Cp Temp hot gas : Subsystem
  Integrator : Integrator  InitialCondition=765+273.15+12  LimitOutput=on  UpperSaturationLimit=1250+273.15  LowerSaturationLimit=600+273.15
  Memory : Memory  InitialCondition=750+273.15
  Scope1 : Scope  Commented=on
  Sum1 : Sum  Inputs=2
  Sum2 : Sum  Inputs=2
  Sum6 : Sum  Inputs=|+-
  time constant : Gain  Gain=1/3.6
  temp gas : Outport
  gas_flow : Outport  Port=2
  wires:
  hot_gas_temp/1 -> Cp Temp hot gas/1(Tinlet), "     4"/2
  hot_gas_flow/1 -> Sum1/1, "     4"/1
  Cp Temp hot gas/1(Cp(T)) -> "     4"/3
  cooling_air_temp/1 -> Cp Temp air/1(Tinlet), "     2"/2
  cooling_air_flow/1 -> Sum1/2, "     2"/1
  Cp Temp air/1(Cp(T)) -> "     2"/3
  "     2"/1 -> Sum2/1
  "     4"/1 -> Sum2/2
  Sum2/1 -> ./1
  Cp Temp/1(Cp(T)) -> "     1"/2
  Memory/1 -> Cp Temp/1(Tinlet)
  "     1"/1 -> ./2
  ./1 -> Sum6/1
  time constant/1 -> Integrator/1
  Sum6/1 -> time constant/1
  Integrator/1 -> temp gas/1, Scope1/1, Sum6/2, Memory/1
  Sum1/1 -> "     1"/1, gas_flow/1

== system AvonGasTurbineDgTwin_fixed/Subsystem/GasGenerator/cooling 2 ==
  cooling_air_temp : Inport
  cooling_air_flow : Inport  Port=2
  hot_gas_flow : Inport  Port=3
  hot_gas_temp : Inport  Port=4
  "     1" : Product  RndMeth=Zero
  "     2" : Product  Inputs=3  RndMeth=Zero
  "     4" : Product  Inputs=3  RndMeth=Zero
  . : Product  Inputs=*/  RndMeth=Zero
  Constant : Constant  Value=-600
  Cp Temp : Subsystem
  Cp Temp air : Subsystem
  Cp Temp hot gas : Subsystem
  Integrator : Integrator  InitialCondition=1204.4  LimitOutput=on  UpperSaturationLimit=2000  LowerSaturationLimit=100
  Memory : Memory  InitialCondition=500+273.15
  Scope1 : Scope  Commented=on
  Scope4 : Scope  Commented=on
  Sum1 : Sum  Inputs=2
  Sum2 : Sum  Inputs=2
  Sum3 : Sum  Inputs=++|
  Sum6 : Sum  Inputs=|+-
  Sum7 : Sum  Inputs=|++
  offset compensator1 : Fcn  Expr=(u-87)/(87)*(14.48)-14.45
  time constant : Gain  Gain=1/5
  gas_flow : Outport
  temp turb : Outport  Port=2
  temp exh turb : Outport  Port=3
  wires:
  Sum6/1 -> time constant/1
  time constant/1 -> Integrator/1
  ./1 -> Sum6/1
  "     1"/1 -> ./2
  Memory/1 -> Cp Temp/1(Tinlet)
  Cp Temp/1(Cp(T)) -> "     1"/2
  Sum1/1 -> Scope4/1, gas_flow/1, "     1"/1, offset compensator1/1
  Sum2/1 -> ./1
  "     4"/1 -> Sum2/2
  "     2"/1 -> Sum2/1
  Cp Temp air/1(Cp(T)) -> "     2"/3
  cooling_air_flow/1 -> "     2"/1, Sum1/2
  cooling_air_temp/1 -> "     2"/2, Cp Temp air/1(Tinlet)
  Cp Temp hot gas/1(Cp(T)) -> "     4"/3
  hot_gas_flow/1 -> "     4"/1, Sum1/1
  hot_gas_temp/1 -> "     4"/2, Cp Temp hot gas/1(Tinlet), Sum3/1
  Integrator/1 -> Sum7/1, Scope1/1, Sum6/2, Memory/1
  Sum3/1 -> temp turb/1
  offset compensator1/1 -> Sum3/2
  Sum7/1 -> temp exh turb/1

== system AvonGasTurbineDgTwin_fixed/Subsystem/GasGenerator/rotor dynamic  ==
  gen_turb : Inport
  consm_comp : Inport  Port=2
  ...1 : Product  Inputs=*/
  ...2 : Product  Inputs=/*
  ...3 : Product
  F1 : Constant  Value=1.9141
  Gain1 : Gain  Gain=0.5
  Gain2 : Gain  Gain=30/pi
  Gain4 : Gain  Gain=pi/30
  Integrator1 : Integrator  InitialCondition=pi/30*7250  LimitOutput=on  UpperSaturationLimit=1200  LowerSaturationLimit=0.01
  J_rotor1 : Gain  Gain=0
  Loss : Gain  Gain=0.001
  Math Function : Math  Operator=square  SignedPower=on
  Memory Omega2 : Memory  InitialCondition=pi/30*7250
  Mux4 : Mux  Inputs=2
  Product2 : Product  Inputs=*/
  Scope1 : Scope  Commented=on
  Scope8 : Scope  Commented=on
  Scope9 : Scope  Commented=on
  Sum1 : Sum  Inputs=++|
  Sum7 : Sum  Inputs=|++
  Sum8 : Sum  Inputs=|+-
  Sum9 : Sum  Inputs=|+-
  freq_rotor2 : Constant
  freq_rotor3 : Constant  Value=7250
  power1 : Constant  Value=7250
  rotor_speed : Outport
  wires:
  F1/1 -> Product2/2
  Memory Omega2/1 -> Sum7/2
  Gain4/1 -> ...2/1, Sum7/1
  Sum7/1 -> ...2/2, ...1/2
  [FG_flow] -> Product2/1
  freq_rotor3/1 -> Gain4/1
  J_rotor1/1 -> Integrator1/1
  Loss/1 -> Sum9/2
  consm_comp/1 -> Sum8/2
  ...2/1 -> Math Function/1
  Math Function/1 -> Loss/1
  power1/1 -> Mux4/2
  Mux4/1 -> Scope9/1
  Gain2/1 -> Mux4/1
  gen_turb/1 -> Sum8/1
  Sum9/1 -> ...1/1
  ...1/1 -> ...3/2
  Product2/1 -> Sum1/1
  Gain1/1 -> Scope1/1, ...3/1
  freq_rotor2/1 -> Sum1/2
  Sum1/1 -> Gain1/1
  ...3/1 -> J_rotor1/1
  Integrator1/1 -> Memory Omega2/1, Gain2/1, rotor_speed/1
  Sum8/1 -> Scope8/1, Sum9/1

== system AvonGasTurbineDgTwin_fixed/Subsystem/PowerTurbine/Cp @ trb. input ==
  Tinlet : Inport
  Cp : Fcn  Expr=(3.355+5.75*1e-4*u(1)-1600*u(1)^(-2))*0.28714  SampleTime=1
  Cp(T) : Outport
  wires:
  Cp/1 -> Cp(T)/1
  Tinlet/1 -> Cp/1

== system AvonGasTurbineDgTwin_fixed/Subsystem/PowerTurbine/Cp @ trb. output ==
  Tinlet : Inport
  Cp : Fcn  Expr=(3.355+5.75*1e-4*u(1)-1600*u(1)^(-2))*0.28714  SampleTime=1
  Cp(T) : Outport
  wires:
  Tinlet/1 -> Cp/1
  Cp/1 -> Cp(T)/1

== system AvonGasTurbineDgTwin_fixed/Subsystem/PowerTurbine/FAULT_28_PTNozzleDamage ==
  hot_gas_flow : Inport
  FAULT_28_multiplier : FromWorkspace  VariableName=FAULT_28_multiplier  SampleTime=-1
  Mux : Mux  Inputs=2
  Product : Product
  Scope{,1..3} (4 alike) : Scope  Commented=on
  Out1 : Outport
  wires:
  FAULT_28_multiplier/1 -> Product/1, Scope/1
  hot_gas_flow/1 -> Scope1/1, Mux/2, Product/2
  Product/1 -> Mux/1, Scope2/1, Out1/1
  Mux/1 -> Scope3/1

== system AvonGasTurbineDgTwin_fixed/Subsystem/PowerTurbine/FAULT_31_PTPowerLoss ==
  In1 : Inport
  FAULT_31_multiplier : FromWorkspace  VariableName=FAULT_31_multiplier  SampleTime=-1
  Mux : Mux  Inputs=2
  Product : Product
  Scope{,1..3} (4 alike) : Scope  Commented=on
  Out1 : Outport
  wires:
  FAULT_31_multiplier/1 -> Product/1, Scope/1
  In1/1 -> Scope1/1, Mux/2, Product/2
  Product/1 -> Mux/1, Scope2/1, Out1/1
  Mux/1 -> Scope3/1

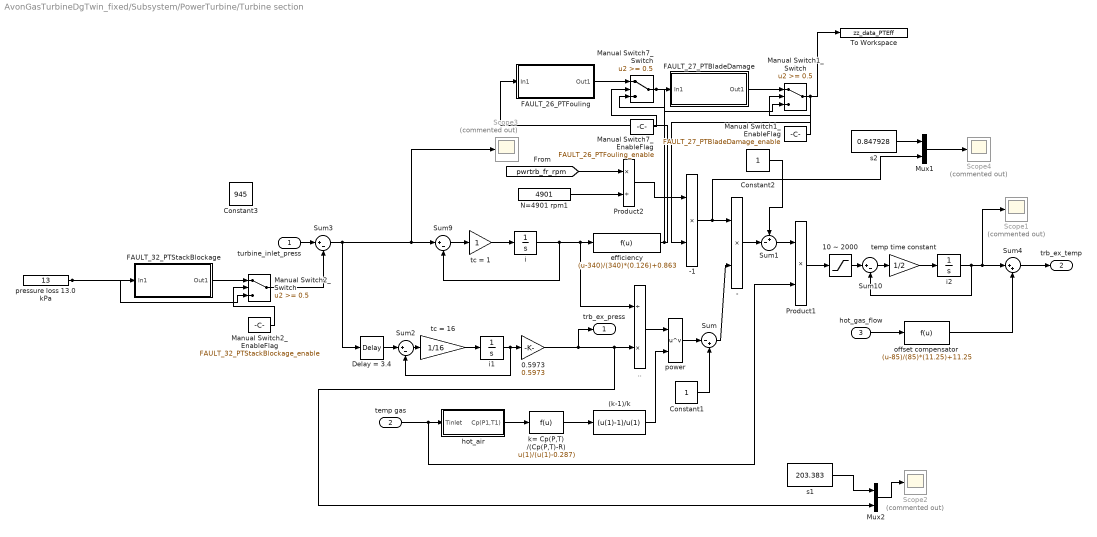
== system AvonGasTurbineDgTwin_fixed/Subsystem/PowerTurbine/Turbine section ==
  turbine_inlet_press : Inport
  temp gas : Inport  Port=2
  hot_gas_flow : Inport  Port=3
  (k-1)/k : Fcn  Expr=(u(1)-1)/u(1)
  - : Product  RndMeth=Zero
  -1 : Product  RndMeth=Zero
  .. : Product  Inputs=/*  RndMeth=Zero
  0.5973 : Gain  Gain=0.5973
  10 ~ 2000 : Saturate  UpperLimit=2000  LowerLimit=10
  Constant1 : Constant
  Constant2 : Constant
  Constant3 : Constant  Value=945
  Delay = 3.4 : TransportDelay  DelayTime=3.4  InitialOutput=230.380
  FAULT_26_PTFouling : Subsystem
  FAULT_27_PTBladeDamage : Subsystem
  FAULT_32_PTStackBlockage : Subsystem
  Manual Switch1_EnableFlag : Constant  Value=FAULT_27_PTBladeDamage_enable
  Manual Switch1_Switch : Switch  Threshold=0.5  SaturateOnIntegerOverflow=off  InputSameDT=off
  Manual Switch2_EnableFlag : Constant  Value=FAULT_32_PTStackBlockage_enable
  Manual Switch2_Switch : Switch  Threshold=0.5  SaturateOnIntegerOverflow=off  InputSameDT=off
  Manual Switch7_EnableFlag : Constant  Value=FAULT_26_PTFouling_enable
  Manual Switch7_Switch : Switch  Threshold=0.5  SaturateOnIntegerOverflow=off  InputSameDT=off
  Mux1 : Mux  Inputs=2
  Mux2 : Mux  Inputs=2
  N=4901 rpm1 : Constant  Value=4901
  Product1 : Product  RndMeth=Zero
  Product2 : Product  Inputs=*/  RndMeth=Zero
  Scope{1..4} (4 alike) : Scope  Commented=on
  Sum : Sum  Inputs=|-+
  Sum1 : Sum  Inputs=+-|
  Sum{2..3,9..10} (4 alike) : Sum  Inputs=|+-
  Sum4 : Sum  Inputs=|++
  To Workspace : ToWorkspace  VariableName=zz_data_PTEff  SampleTime=0.2
  efficiency : Fcn  Expr=(u-340)/(340)*(0.126)+0.863
  hot_air : Subsystem
  i : Integrator  InitialCondition=340  LimitOutput=on  UpperSaturationLimit=1000  LowerSaturationLimit=1
  i1 : Integrator  InitialCondition=203  LimitOutput=on  UpperSaturationLimit=500  LowerSaturationLimit=1
  i2 : Integrator  InitialCondition=1082  LimitOutput=on  UpperSaturationLimit=2000  LowerSaturationLimit=400
  k= Cp(P,T) /(Cp(P,T)-R) : Fcn  Expr=u(1)/(u(1)-0.287)
  offset compensator : Fcn  Expr=(u-85)/(85)*(11.25)+11.25  SampleTime=1
  power : Math  Operator=pow  SignedPower=on
  pressure loss 13.0 kPa : Constant  Value=13
  s1 : Constant  Value=203.383
  s2 : Constant  Value=0.847928
  tc = 1 : Gain
  tc = 16 : Gain  Gain=1/16
  temp time constant : Gain  Gain=1/2
  trb_ex_press : Outport
  trb_ex_temp : Outport  Port=2
  wires:
  ../1 -> power/1
  turbine_inlet_press/1 -> Sum3/1
  tc = 16/1 -> i1/1
  Sum2/1 -> tc = 16/1
  i1/1 -> 0.5973/1, Sum2/2
  s2/1 -> Mux1/1
  Mux1/1 -> Scope4/1
  i2/1 -> Sum10/2, Sum4/1, Scope1/1
  10 ~ 2000/1 -> Sum10/1
  temp gas/1 -> hot_air/1(Tinlet), Product1/2
  Sum1/1 -> Product1/1
  Constant2/1 -> Sum1/1
  Product1/1 -> 10 ~ 2000/1
  temp time constant/1 -> i2/1
  Sum10/1 -> temp time constant/1
  tc = 1/1 -> i/1
  Sum9/1 -> tc = 1/1
  Sum/1 -> -/2
  (k-1)/k/1 -> power/2
  hot_air/1(Cp(P1,T1)) -> k= Cp(P,T) /(Cp(P,T)-R)/1
  k= Cp(P,T) /(Cp(P,T)-R)/1 -> (k-1)/k/1
  Sum3/1 -> Sum9/1, Scope3/1, Delay = 3.4/1
  -/1 -> Sum1/2
  Constant1/1 -> Sum/2
  power/1 -> Sum/1
  i/1 -> efficiency/1, ../1, Sum9/2
  s1/1 -> Mux2/1
  Mux2/1 -> Scope2/1
  offset compensator/1 -> Sum4/2
  hot_gas_flow/1 -> offset compensator/1
  Sum4/1 -> trb_ex_temp/1
  0.5973/1 -> trb_ex_press/1, Mux2/2, ../2
  N=4901 rpm1/1 -> Product2/2
  [pwrtrb_fr_rpm] -> Product2/1
  Product2/1 -> -1/1
  -1/1 -> Mux1/2, -/1
  Delay = 3.4/1 -> Sum2/1
  efficiency/1 -> FAULT_26_PTFouling/1(In1), Manual Switch7_Switch/3
  pressure loss 13.0 kPa/1 -> FAULT_32_PTStackBlockage/1(In1), Manual Switch2_Switch/3
  FAULT_27_PTBladeDamage/1(Out1) -> Manual Switch1_Switch/1
  Manual Switch1_EnableFlag/1 -> Manual Switch1_Switch/2
  Manual Switch1_Switch/1 -> To Workspace/1, -1/2
  FAULT_32_PTStackBlockage/1(Out1) -> Manual Switch2_Switch/1
  Manual Switch2_EnableFlag/1 -> Manual Switch2_Switch/2
  Manual Switch2_Switch/1 -> Sum3/2
  FAULT_26_PTFouling/1(Out1) -> Manual Switch7_Switch/1
  Manual Switch7_EnableFlag/1 -> Manual Switch7_Switch/2
  Manual Switch7_Switch/1 -> Manual Switch1_Switch/3, FAULT_27_PTBladeDamage/1(In1)

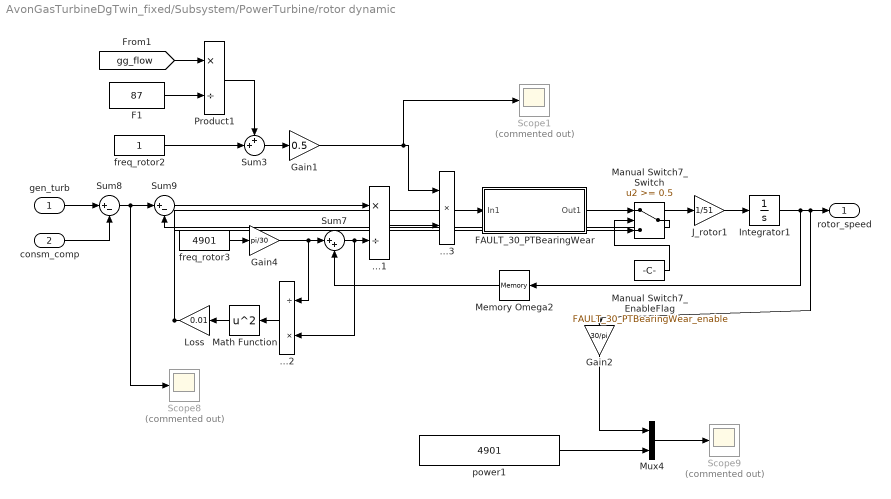
== system AvonGasTurbineDgTwin_fixed/Subsystem/PowerTurbine/rotor dynamic ==
  gen_turb : Inport
  consm_comp : Inport  Port=2
  ...1 : Product  Inputs=*/
  ...2 : Product  Inputs=/*
  ...3 : Product
  F1 : Constant  Value=87
  FAULT_30_PTBearingWear : Subsystem
  Gain1 : Gain  Gain=0.5
  Gain2 : Gain  Gain=30/pi
  Gain4 : Gain  Gain=pi/30
  Integrator1 : Integrator  InitialCondition=pi/30*4901  LimitOutput=on  UpperSaturationLimit=4900*1.20*pi/30  LowerSaturationLimit=0.01
  J_rotor1 : Gain  Gain=1/51
  Loss : Gain  Gain=0.01
  Manual Switch7_EnableFlag : Constant  Value=FAULT_30_PTBearingWear_enable
  Manual Switch7_Switch : Switch  Threshold=0.5  SaturateOnIntegerOverflow=off  InputSameDT=off
  Math Function : Math  Operator=square  SignedPower=on
  Memory Omega2 : Memory  InitialCondition=pi/30*4901
  Mux4 : Mux  Inputs=2
  Product1 : Product  Inputs=*/
  Scope1 : Scope  Commented=on
  Scope8 : Scope  Commented=on
  Scope9 : Scope  Commented=on
  Sum3 : Sum  Inputs=++|
  Sum7 : Sum  Inputs=|++
  Sum8 : Sum  Inputs=|+-
  Sum9 : Sum  Inputs=|+-
  freq_rotor2 : Constant
  freq_rotor3 : Constant  Value=4901
  power1 : Constant  Value=4901
  rotor_speed : Outport
  wires:
  Sum9/1 -> ...1/1
  Memory Omega2/1 -> Sum7/2
  Gain4/1 -> ...2/1, Sum7/1
  Sum7/1 -> ...2/2, ...1/2
  ...1/1 -> ...3/2
  J_rotor1/1 -> Integrator1/1
  consm_comp/1 -> Sum8/2
  Sum8/1 -> Scope8/1, Sum9/1
  ...2/1 -> Math Function/1
  Gain1/1 -> ...3/1, Scope1/1
  Math Function/1 -> Loss/1
  Integrator1/1 -> Memory Omega2/1, rotor_speed/1, Gain2/1
  power1/1 -> Mux4/2
  Mux4/1 -> Scope9/1
  Gain2/1 -> Mux4/1
  gen_turb/1 -> Sum8/1
  freq_rotor3/1 -> Gain4/1
  F1/1 -> Product1/2
  [gg_flow] -> Product1/1
  Product1/1 -> Sum3/1
  freq_rotor2/1 -> Sum3/2
  Sum3/1 -> Gain1/1
  FAULT_30_PTBearingWear/1(Out1) -> Manual Switch7_Switch/1
  Manual Switch7_EnableFlag/1 -> Manual Switch7_Switch/2
  Loss/1 -> FAULT_30_PTBearingWear/1(In1), Manual Switch7_Switch/3
  Manual Switch7_Switch/1 -> Sum9/2
  ...3/1 -> J_rotor1/1

== system AvonGasTurbineDgTwin_fixed/Subsystem/comp_temp1/Air_Intake ==
  In1 : Inport
  Filter Constant : Constant  Value=0.0003
  Product : Product
  Scope : Scope  Commented=on
  Square : Math  Operator=square
  deltaP : Outport
  wires:
  In1/1 -> Square/1
  Filter Constant/1 -> Product/1
  Square/1 -> Scope/1, Product/2
  Product/1 -> deltaP/1

== system AvonGasTurbineDgTwin_fixed/Subsystem/comp_temp1/Cp @Cop Outlet ==
  Tinlet : Inport
  Cp : Fcn  Expr=(3.355+5.75*1e-4*u(1)-1600*u(1)^(-2))*0.28714  SampleTime=1
  oC-----> K : Fcn  Expr=(u(1)+273.15)  SampleTime=1
  Cp(T) : Outport
  wires:
  oC-----> K/1 -> Cp/1
  Cp/1 -> Cp(T)/1
  Tinlet/1 -> oC-----> K/1

== system AvonGasTurbineDgTwin_fixed/Subsystem/comp_temp1/Cp_com_in ==
  humidity ratio : Inport
  pressuer : Inport  Port=2
  temp. : Inport  Port=3
  .1 : Product  RndMeth=Zero
  .2 : Product  RndMeth=Zero
  Cp dry air : Subsystem
  Cp steam : Subsystem
  R dry air : Constant  Value=0.287
  R steam : Constant  Value=0.4615
  Specific humidity : Subsystem
  Sum1 : Sum  Inputs=++|
  Sum4 : Sum  Inputs=|++
  Cp : Outport
  Rwet : Outport  Port=2
  wires:
  .1/1 -> Sum4/1
  Specific humidity/1(y) -> .2/2, .1/1
  Cp steam/1(Cp(T)) -> .1/2
  Cp dry air/1(Cp(T)) -> Sum4/2
  humidity ratio/1 -> Specific humidity/1(humidity)
  pressuer/1 -> Specific humidity/2(Press_kPa)
  Sum4/1 -> Cp/1
  temp./1 -> Specific humidity/3(temp), Cp steam/1(Tinlet), Cp dry air/1(Tinlet)
  R steam/1 -> .2/1
  .2/1 -> Sum1/2
  Sum1/1 -> Rwet/1
  R dry air/1 -> Sum1/1

== system AvonGasTurbineDgTwin_fixed/Subsystem/comp_temp1/FAULT_01_AirIntakeFilterFouling ==
  deltaP : Inport
  FAULT_01_multiplier : FromWorkspace  VariableName=FAULT_01_multiplier  SampleTime=-1
  Mux : Mux  Inputs=2
  Product : Product
  Scope{,1..3} (4 alike) : Scope  Commented=on
  Out1 : Outport
  wires:
  FAULT_01_multiplier/1 -> Product/1, Scope/1
  deltaP/1 -> Scope1/1, Mux/2, Product/2
  Product/1 -> Mux/1, Scope2/1, Out1/1
  Mux/1 -> Scope3/1

== system AvonGasTurbineDgTwin_fixed/Subsystem/comp_temp1/FAULT_02_CompBladeFouling ==
  In1 : Inport
  FAULT_02_multiplier : FromWorkspace  VariableName=FAULT_02_multiplier  SampleTime=-1
  Mux : Mux  Inputs=2
  Product : Product
  Scope{,1..3} (4 alike) : Scope  Commented=on
  Out1 : Outport
  wires:
  FAULT_02_multiplier/1 -> Product/1, Scope/1
  In1/1 -> Scope1/1, Mux/2, Product/2
  Product/1 -> Mux/1, Scope2/1, Out1/1
  Mux/1 -> Scope3/1

== system AvonGasTurbineDgTwin_fixed/Subsystem/comp_temp1/FAULT_03_CompBladeDamage ==
  In1 : Inport
  FAULT_03_multiplier : FromWorkspace  VariableName=FAULT_03_multiplier  SampleTime=-1
  Mux : Mux  Inputs=2
  Product : Product
  Scope{,1..3} (4 alike) : Scope  Commented=on
  Out1 : Outport
  wires:
  FAULT_03_multiplier/1 -> Product/1, Scope/1
  In1/1 -> Scope1/1, Mux/2, Product/2
  Product/1 -> Mux/1, Scope2/1, Out1/1
  Mux/1 -> Scope3/1

== system AvonGasTurbineDgTwin_fixed/Subsystem/comp_temp1/FAULT_04_CompSurgeStall ==
  In1 : Inport
  FAULT_04_multiplier : FromWorkspace  VariableName=FAULT_04_multiplier  SampleTime=-1
  Mux : Mux  Inputs=2
  Product : Product
  Scope{,1..3} (4 alike) : Scope  Commented=on
  Out1 : Outport
  wires:
  FAULT_04_multiplier/1 -> Product/1, Scope/1
  In1/1 -> Scope1/1, Mux/2, Product/2
  Product/1 -> Mux/1, Scope2/1, Out1/1
  Mux/1 -> Scope3/1

== system AvonGasTurbineDgTwin_fixed/Subsystem/comp_temp1/FAULT_05_DiffuserDamage ==
  In1 : Inport
  FAULT_05_multiplier : FromWorkspace  VariableName=FAULT_05_multiplier  SampleTime=-1
  Mux : Mux  Inputs=2
  Product : Product
  Scope{,1..3} (4 alike) : Scope  Commented=on
  Out1 : Outport
  wires:
  FAULT_05_multiplier/1 -> Product/1, Scope/1
  In1/1 -> Scope1/1, Mux/2, Product/2
  Product/1 -> Mux/1, Scope2/1, Out1/1
  Mux/1 -> Scope3/1

== system AvonGasTurbineDgTwin_fixed/Subsystem/Combustor1/combustion chamber 1/ Cp dry air  ==
  Tinlet : Inport
  Cp : Fcn  Expr=(3.355+5.75*1e-4*u(1)-1600*u(1)^(-2))*0.28714  SampleTime=1
  Cp(T) : Outport
  wires:
  Tinlet/1 -> Cp/1
  Cp/1 -> Cp(T)/1

== system AvonGasTurbineDgTwin_fixed/Subsystem/Combustor1/combustion chamber 1/Cp Hot Gas  ==
  Tinlet : Inport
  Cp : Fcn  Expr=(3.355+5.75*1e-4*u(1)-1600*u(1)^(-2))*0.28714  SampleTime=1
  Cp(T) : Outport
  wires:
  Tinlet/1 -> Cp/1  "Kelvin"
  Cp/1 -> Cp(T)/1
